simulink model "RoverPlatformArch"  (R2026a)
settings: Solver=VariableStepAuto
settings Model: DataDictionary=RoverPlatformInterfaces.sldd  Creator=potlo  LastModifiedBy=potlo

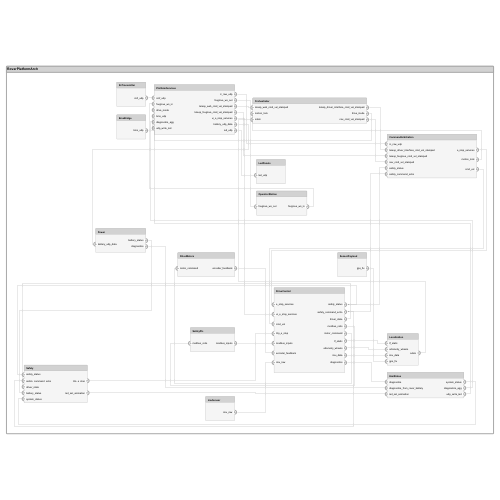
[thumbnail: Simulink's stored preview of the top-level diagram]
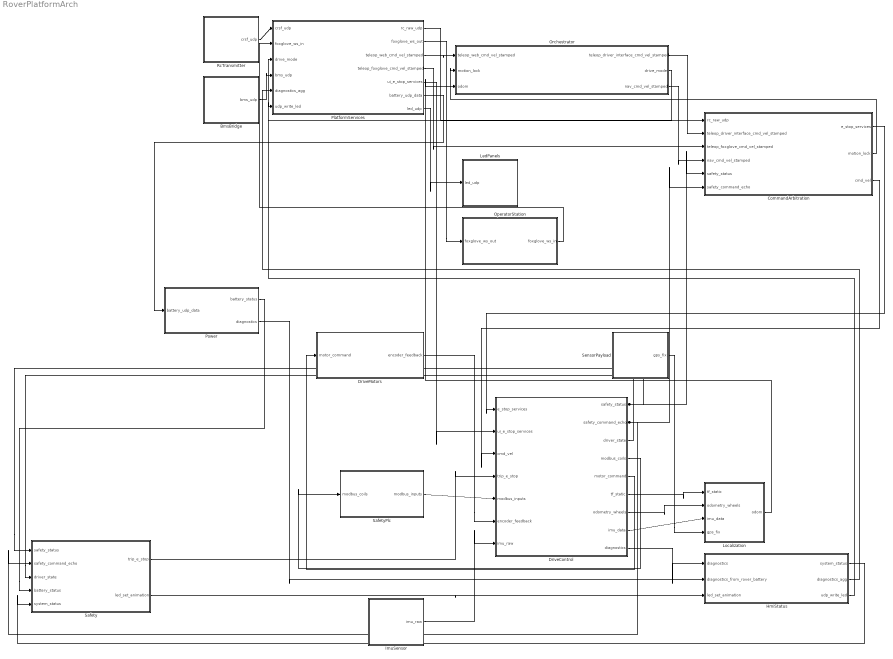
== system RoverPlatformArch ==
  BmsBridge : Subsystem
      settings: PortSchema="{\"entries\":[{\"content\":{\"headerSize\":26,\"margin\":15,\"minimumSpacing\":25,\"sides\":[{\"content\":{},\"type\":\"ConnectorPlacement.EquallySpacedRectSide\",\"uuid\":\"6054c9f0-8412-410d-9e26-05323c576afd\"},{\"content\":{\"connectorIds\":[\"Out1\"],\"side\":\"RIGHT\"},\"type\":\"ConnectorPlacement.EquallySpacedRectSide\",\"uuid\":\"23d80627-c7f5-467f-845e-39a8ba0f8903\"},{\"content\":{\"side\":\"TOP\"},\"type\":\"ConnectorPlacement.EquallySpacedRectSide\",\"uuid\":\"85f79d16-0e4c-46b5-a9e4-5492e918629f\"}]},\"type\":\"ConnectorPlacement.EquallySpacedConnector\",\"uuid\":\"014a8f15-8cf2-4a07-97a2-6bf2fab6c72b\"}],\"packageUris\":[\"http://schema.mathworks.com/mf0/Connector/R2020b\"],\"version\":\"1.0\"}"
  CommandArbitration : Subsystem
      settings: PortSchema="{\"entries\":[{\"content\":{\"headerSize\":26,\"margin\":15,\"minimumSpacing\":25,\"sides\":[{\"content\":{\"connectorIds\":[\"In1\",\"In2\",\"In3\",\"In4\",\"In5\",\"In6\"]},\"type\":\"ConnectorPlacement.EquallySpacedRectSide\",\"uuid\":\"6054c9f0-8412-410d-9e26-05323c576afd\"},{\"content\":{\"connectorIds\":[\"Out1\",\"Out2\",\"Out3\"],\"side\":\"RIGHT\"},\"type\":\"ConnectorPlacement.EquallySpacedRectSide\",\"uuid\":\"23d80627-c7f5-467f-845e-39a8ba0f8903\"},{\"content\":{\"side\":\"TOP\"},\"type\":\"ConnectorPlacement.EquallySpacedRectSide\",\"uuid\":\"85f79d16-0e4c-46b5-a9e4-5492e918629f\"}]},\"type\":\"ConnectorPlacement.EquallySpacedConnector\",\"uuid\":\"014a8f15-8cf2-4a07-97a2-6bf2fab6c72b\"}],\"packageUris\":[\"http://schema.mathworks.com/mf0/Connector/R2020b\"],\"version\":\"1.0\"}"
  DriveControl : Subsystem
      settings: PortSchema="{\"entries\":[{\"content\":{\"headerSize\":26,\"margin\":15,\"minimumSpacing\":25,\"sides\":[{\"content\":{\"connectorIds\":[\"In1\",\"In2\",\"In3\",\"In4\",\"In5\",\"In6\",\"In7\"]},\"type\":\"ConnectorPlacement.EquallySpacedRectSide\",\"uuid\":\"6054c9f0-8412-410d-9e26-05323c576afd\"},{\"content\":{\"connectorIds\":[\"Out1\",\"Out2\",\"Out3\",\"Out4\",\"Out5\",\"Out6\",\"Out7\",\"Out8\",\"Out9\"],\"side\":\"RIGHT\"},\"type\":\"ConnectorPlacement.EquallySpacedRectSide\",\"uuid\":\"23d80627-c7f5-467f-845e-39a8ba0f8903\"},{\"content\":{\"side\":\"TOP\"},\"type\":\"ConnectorPlacement.EquallySpacedRectSide\",\"uuid\":\"85f79d16-0e4c-46b5-a9e4-5492e918629f\"}]},\"type\":\"ConnectorPlacement.EquallySpacedConnector\",\"uuid\":\"014a8f15-8cf2-4a07-97a2-6bf2fab6c72b\"}],\"packageUris\":[\"http://schema.mathworks.com/mf0/Connector/R2020b\"],\"version\":\"1.0\"}"
  DriveMotors : Subsystem
      settings: PortSchema="{\"entries\":[{\"content\":{\"headerSize\":26,\"margin\":15,\"minimumSpacing\":25,\"sides\":[{\"content\":{\"connectorIds\":[\"In1\"]},\"type\":\"ConnectorPlacement.EquallySpacedRectSide\",\"uuid\":\"6054c9f0-8412-410d-9e26-05323c576afd\"},{\"content\":{\"connectorIds\":[\"Out1\"],\"side\":\"RIGHT\"},\"type\":\"ConnectorPlacement.EquallySpacedRectSide\",\"uuid\":\"23d80627-c7f5-467f-845e-39a8ba0f8903\"},{\"content\":{\"side\":\"TOP\"},\"type\":\"ConnectorPlacement.EquallySpacedRectSide\",\"uuid\":\"85f79d16-0e4c-46b5-a9e4-5492e918629f\"}]},\"type\":\"ConnectorPlacement.EquallySpacedConnector\",\"uuid\":\"014a8f15-8cf2-4a07-97a2-6bf2fab6c72b\"}],\"packageUris\":[\"http://schema.mathworks.com/mf0/Connector/R2020b\"],\"version\":\"1.0\"}"
  HmiStatus : Subsystem
      settings: PortSchema="{\"entries\":[{\"content\":{\"headerSize\":26,\"margin\":15,\"minimumSpacing\":25,\"sides\":[{\"content\":{\"connectorIds\":[\"In1\",\"In2\",\"In3\"]},\"type\":\"ConnectorPlacement.EquallySpacedRectSide\",\"uuid\":\"6054c9f0-8412-410d-9e26-05323c576afd\"},{\"content\":{\"connectorIds\":[\"Out1\",\"Out2\",\"Out3\"],\"side\":\"RIGHT\"},\"type\":\"ConnectorPlacement.EquallySpacedRectSide\",\"uuid\":\"23d80627-c7f5-467f-845e-39a8ba0f8903\"},{\"content\":{\"side\":\"TOP\"},\"type\":\"ConnectorPlacement.EquallySpacedRectSide\",\"uuid\":\"85f79d16-0e4c-46b5-a9e4-5492e918629f\"}]},\"type\":\"ConnectorPlacement.EquallySpacedConnector\",\"uuid\":\"014a8f15-8cf2-4a07-97a2-6bf2fab6c72b\"}],\"packageUris\":[\"http://schema.mathworks.com/mf0/Connector/R2020b\"],\"version\":\"1.0\"}"
  ImuSensor : Subsystem
      settings: PortSchema="{\"entries\":[{\"content\":{\"headerSize\":26,\"margin\":15,\"minimumSpacing\":25,\"sides\":[{\"content\":{},\"type\":\"ConnectorPlacement.EquallySpacedRectSide\",\"uuid\":\"6054c9f0-8412-410d-9e26-05323c576afd\"},{\"content\":{\"connectorIds\":[\"Out1\"],\"side\":\"RIGHT\"},\"type\":\"ConnectorPlacement.EquallySpacedRectSide\",\"uuid\":\"23d80627-c7f5-467f-845e-39a8ba0f8903\"},{\"content\":{\"side\":\"TOP\"},\"type\":\"ConnectorPlacement.EquallySpacedRectSide\",\"uuid\":\"85f79d16-0e4c-46b5-a9e4-5492e918629f\"}]},\"type\":\"ConnectorPlacement.EquallySpacedConnector\",\"uuid\":\"014a8f15-8cf2-4a07-97a2-6bf2fab6c72b\"}],\"packageUris\":[\"http://schema.mathworks.com/mf0/Connector/R2020b\"],\"version\":\"1.0\"}"
  LedPanels : Subsystem
      settings: PortSchema="{\"entries\":[{\"content\":{\"headerSize\":26,\"margin\":15,\"minimumSpacing\":25,\"sides\":[{\"content\":{\"connectorIds\":[\"In1\"]},\"type\":\"ConnectorPlacement.EquallySpacedRectSide\",\"uuid\":\"6054c9f0-8412-410d-9e26-05323c576afd\"},{\"content\":{\"side\":\"RIGHT\"},\"type\":\"ConnectorPlacement.EquallySpacedRectSide\",\"uuid\":\"23d80627-c7f5-467f-845e-39a8ba0f8903\"},{\"content\":{\"side\":\"TOP\"},\"type\":\"ConnectorPlacement.EquallySpacedRectSide\",\"uuid\":\"85f79d16-0e4c-46b5-a9e4-5492e918629f\"}]},\"type\":\"ConnectorPlacement.EquallySpacedConnector\",\"uuid\":\"014a8f15-8cf2-4a07-97a2-6bf2fab6c72b\"}],\"packageUris\":[\"http://schema.mathworks.com/mf0/Connector/R2020b\"],\"version\":\"1.0\"}"
  Localization : Subsystem
      settings: PortSchema="{\"entries\":[{\"content\":{\"headerSize\":26,\"margin\":15,\"minimumSpacing\":25,\"sides\":[{\"content\":{\"connectorIds\":[\"In1\",\"In2\",\"In3\",\"In4\"]},\"type\":\"ConnectorPlacement.EquallySpacedRectSide\",\"uuid\":\"6054c9f0-8412-410d-9e26-05323c576afd\"},{\"content\":{\"connectorIds\":[\"Out1\"],\"side\":\"RIGHT\"},\"type\":\"ConnectorPlacement.EquallySpacedRectSide\",\"uuid\":\"23d80627-c7f5-467f-845e-39a8ba0f8903\"},{\"content\":{\"side\":\"TOP\"},\"type\":\"ConnectorPlacement.EquallySpacedRectSide\",\"uuid\":\"85f79d16-0e4c-46b5-a9e4-5492e918629f\"}]},\"type\":\"ConnectorPlacement.EquallySpacedConnector\",\"uuid\":\"014a8f15-8cf2-4a07-97a2-6bf2fab6c72b\"}],\"packageUris\":[\"http://schema.mathworks.com/mf0/Connector/R2020b\"],\"version\":\"1.0\"}"
  OperatorStation : Subsystem
      settings: PortSchema="{\"entries\":[{\"content\":{\"headerSize\":26,\"margin\":15,\"minimumSpacing\":25,\"sides\":[{\"content\":{\"connectorIds\":[\"In1\"]},\"type\":\"ConnectorPlacement.EquallySpacedRectSide\",\"uuid\":\"6054c9f0-8412-410d-9e26-05323c576afd\"},{\"content\":{\"connectorIds\":[\"Out1\"],\"side\":\"RIGHT\"},\"type\":\"ConnectorPlacement.EquallySpacedRectSide\",\"uuid\":\"23d80627-c7f5-467f-845e-39a8ba0f8903\"},{\"content\":{\"side\":\"TOP\"},\"type\":\"ConnectorPlacement.EquallySpacedRectSide\",\"uuid\":\"85f79d16-0e4c-46b5-a9e4-5492e918629f\"}]},\"type\":\"ConnectorPlacement.EquallySpacedConnector\",\"uuid\":\"014a8f15-8cf2-4a07-97a2-6bf2fab6c72b\"}],\"packageUris\":[\"http://schema.mathworks.com/mf0/Connector/R2020b\"],\"version\":\"1.0\"}"
  Orchestrator : Subsystem
      settings: PortSchema="{\"entries\":[{\"content\":{\"headerSize\":26,\"margin\":15,\"minimumSpacing\":25,\"sides\":[{\"content\":{\"connectorIds\":[\"In1\",\"In2\",\"In3\"]},\"type\":\"ConnectorPlacement.EquallySpacedRectSide\",\"uuid\":\"6054c9f0-8412-410d-9e26-05323c576afd\"},{\"content\":{\"connectorIds\":[\"Out1\",\"Out2\",\"Out3\"],\"side\":\"RIGHT\"},\"type\":\"ConnectorPlacement.EquallySpacedRectSide\",\"uuid\":\"23d80627-c7f5-467f-845e-39a8ba0f8903\"},{\"content\":{\"side\":\"TOP\"},\"type\":\"ConnectorPlacement.EquallySpacedRectSide\",\"uuid\":\"85f79d16-0e4c-46b5-a9e4-5492e918629f\"}]},\"type\":\"ConnectorPlacement.EquallySpacedConnector\",\"uuid\":\"014a8f15-8cf2-4a07-97a2-6bf2fab6c72b\"}],\"packageUris\":[\"http://schema.mathworks.com/mf0/Connector/R2020b\"],\"version\":\"1.0\"}"
  PlatformServices : Subsystem
      settings: PortSchema="{\"entries\":[{\"content\":{\"headerSize\":26,\"margin\":15,\"minimumSpacing\":25,\"sides\":[{\"content\":{\"connectorIds\":[\"In1\",\"In2\",\"In3\",\"In4\",\"In5\",\"In6\"]},\"type\":\"ConnectorPlacement.EquallySpacedRectSide\",\"uuid\":\"6054c9f0-8412-410d-9e26-05323c576afd\"},{\"content\":{\"connectorIds\":[\"Out1\",\"Out2\",\"Out3\",\"Out4\",\"Out5\",\"Out6\",\"Out7\"],\"side\":\"RIGHT\"},\"type\":\"ConnectorPlacement.EquallySpacedRectSide\",\"uuid\":\"23d80627-c7f5-467f-845e-39a8ba0f8903\"},{\"content\":{\"side\":\"TOP\"},\"type\":\"ConnectorPlacement.EquallySpacedRectSide\",\"uuid\":\"85f79d16-0e4c-46b5-a9e4-5492e918629f\"}]},\"type\":\"ConnectorPlacement.EquallySpacedConnector\",\"uuid\":\"014a8f15-8cf2-4a07-97a2-6bf2fab6c72b\"}],\"packageUris\":[\"http://schema.mathworks.com/mf0/Connector/R2020b\"],\"version\":\"1.0\"}"
  Power : Subsystem
      settings: PortSchema="{\"entries\":[{\"content\":{\"headerSize\":26,\"margin\":15,\"minimumSpacing\":25,\"sides\":[{\"content\":{\"connectorIds\":[\"In1\"]},\"type\":\"ConnectorPlacement.EquallySpacedRectSide\",\"uuid\":\"6054c9f0-8412-410d-9e26-05323c576afd\"},{\"content\":{\"connectorIds\":[\"Out1\",\"Out2\"],\"side\":\"RIGHT\"},\"type\":\"ConnectorPlacement.EquallySpacedRectSide\",\"uuid\":\"23d80627-c7f5-467f-845e-39a8ba0f8903\"},{\"content\":{\"side\":\"TOP\"},\"type\":\"ConnectorPlacement.EquallySpacedRectSide\",\"uuid\":\"85f79d16-0e4c-46b5-a9e4-5492e918629f\"}]},\"type\":\"ConnectorPlacement.EquallySpacedConnector\",\"uuid\":\"014a8f15-8cf2-4a07-97a2-6bf2fab6c72b\"}],\"packageUris\":[\"http://schema.mathworks.com/mf0/Connector/R2020b\"],\"version\":\"1.0\"}"
  RcTransmitter : Subsystem
      settings: PortSchema="{\"entries\":[{\"content\":{\"headerSize\":26,\"margin\":15,\"minimumSpacing\":25,\"sides\":[{\"content\":{},\"type\":\"ConnectorPlacement.EquallySpacedRectSide\",\"uuid\":\"6054c9f0-8412-410d-9e26-05323c576afd\"},{\"content\":{\"connectorIds\":[\"Out1\"],\"side\":\"RIGHT\"},\"type\":\"ConnectorPlacement.EquallySpacedRectSide\",\"uuid\":\"23d80627-c7f5-467f-845e-39a8ba0f8903\"},{\"content\":{\"side\":\"TOP\"},\"type\":\"ConnectorPlacement.EquallySpacedRectSide\",\"uuid\":\"85f79d16-0e4c-46b5-a9e4-5492e918629f\"}]},\"type\":\"ConnectorPlacement.EquallySpacedConnector\",\"uuid\":\"014a8f15-8cf2-4a07-97a2-6bf2fab6c72b\"}],\"packageUris\":[\"http://schema.mathworks.com/mf0/Connector/R2020b\"],\"version\":\"1.0\"}"
  Safety : Subsystem
      settings: PortSchema="{\"entries\":[{\"content\":{\"headerSize\":26,\"margin\":15,\"minimumSpacing\":25,\"sides\":[{\"content\":{\"connectorIds\":[\"In1\",\"In2\",\"In3\",\"In4\",\"In5\"]},\"type\":\"ConnectorPlacement.EquallySpacedRectSide\",\"uuid\":\"6054c9f0-8412-410d-9e26-05323c576afd\"},{\"content\":{\"connectorIds\":[\"Out1\",\"Out2\"],\"side\":\"RIGHT\"},\"type\":\"ConnectorPlacement.EquallySpacedRectSide\",\"uuid\":\"23d80627-c7f5-467f-845e-39a8ba0f8903\"},{\"content\":{\"side\":\"TOP\"},\"type\":\"ConnectorPlacement.EquallySpacedRectSide\",\"uuid\":\"85f79d16-0e4c-46b5-a9e4-5492e918629f\"}]},\"type\":\"ConnectorPlacement.EquallySpacedConnector\",\"uuid\":\"014a8f15-8cf2-4a07-97a2-6bf2fab6c72b\"}],\"packageUris\":[\"http://schema.mathworks.com/mf0/Connector/R2020b\"],\"version\":\"1.0\"}"
  SafetyPlc : Subsystem
      settings: PortSchema="{\"entries\":[{\"content\":{\"headerSize\":26,\"margin\":15,\"minimumSpacing\":25,\"sides\":[{\"content\":{\"connectorIds\":[\"In1\"]},\"type\":\"ConnectorPlacement.EquallySpacedRectSide\",\"uuid\":\"6054c9f0-8412-410d-9e26-05323c576afd\"},{\"content\":{\"connectorIds\":[\"Out1\"],\"side\":\"RIGHT\"},\"type\":\"ConnectorPlacement.EquallySpacedRectSide\",\"uuid\":\"23d80627-c7f5-467f-845e-39a8ba0f8903\"},{\"content\":{\"side\":\"TOP\"},\"type\":\"ConnectorPlacement.EquallySpacedRectSide\",\"uuid\":\"85f79d16-0e4c-46b5-a9e4-5492e918629f\"}]},\"type\":\"ConnectorPlacement.EquallySpacedConnector\",\"uuid\":\"014a8f15-8cf2-4a07-97a2-6bf2fab6c72b\"}],\"packageUris\":[\"http://schema.mathworks.com/mf0/Connector/R2020b\"],\"version\":\"1.0\"}"
  SensorPayload : Subsystem
      settings: PortSchema="{\"entries\":[{\"content\":{\"headerSize\":26,\"margin\":15,\"minimumSpacing\":25,\"sides\":[{\"content\":{},\"type\":\"ConnectorPlacement.EquallySpacedRectSide\",\"uuid\":\"6054c9f0-8412-410d-9e26-05323c576afd\"},{\"content\":{\"connectorIds\":[\"Out1\"],\"side\":\"RIGHT\"},\"type\":\"ConnectorPlacement.EquallySpacedRectSide\",\"uuid\":\"23d80627-c7f5-467f-845e-39a8ba0f8903\"},{\"content\":{\"side\":\"TOP\"},\"type\":\"ConnectorPlacement.EquallySpacedRectSide\",\"uuid\":\"85f79d16-0e4c-46b5-a9e4-5492e918629f\"}]},\"type\":\"ConnectorPlacement.EquallySpacedConnector\",\"uuid\":\"014a8f15-8cf2-4a07-97a2-6bf2fab6c72b\"}],\"packageUris\":[\"http://schema.mathworks.com/mf0/Connector/R2020b\"],\"version\":\"1.0\"}"
  wires:
  PlatformServices/4(teleop_foxglove_cmd_vel_stamped) -> CommandArbitration/3(teleop_foxglove_cmd_vel_stamped)
  RcTransmitter/1(crsf_udp) -> PlatformServices/1(crsf_udp)
  Power/1(battery_status) -> Safety/4(battery_status)
  HmiStatus/1(system_status) -> Safety/5(system_status)
  Safety/1(trip_e_stop) -> DriveControl/4(trip_e_stop)
  Power/2(diagnostics) -> HmiStatus/2(diagnostics_from_rover_battery)
  Safety/2(led_set_animation) -> HmiStatus/3(led_set_animation)
  BmsBridge/1(bms_udp) -> PlatformServices/4(bms_udp)
  PlatformServices/1(rc_raw_udp) -> CommandArbitration/1(rc_raw_udp)
  DriveControl/7(odometry_wheels) -> Localization/2(odometry_wheels)
  PlatformServices/2(foxglove_ws_out) -> OperatorStation/1(foxglove_ws_out)
  PlatformServices/3(teleop_web_cmd_vel_stamped) -> Orchestrator/1(teleop_web_cmd_vel_stamped)
  PlatformServices/5(ui_e_stop_services) -> DriveControl/2(ui_e_stop_services)
  PlatformServices/6(battery_udp_data) -> Power/1(battery_udp_data)
  PlatformServices/7(led_udp) -> LedPanels/1(led_udp)
  DriveMotors/1(encoder_feedback) -> DriveControl/6(encoder_feedback)
  SafetyPlc/1(modbus_inputs) -> DriveControl/5(modbus_inputs)
  DriveControl/1(safety_status) -> Safety/1(safety_status), CommandArbitration/5(safety_status)
  ImuSensor/1(imu_raw) -> DriveControl/7(imu_raw)
  SensorPayload/1(gps_fix) -> Localization/4(gps_fix)
  Orchestrator/1(teleop_driver_interface_cmd_vel_stamped) -> CommandArbitration/2(teleop_driver_interface_cmd_vel_stamped)
  Localization/1(odom) -> Orchestrator/3(odom)
  Orchestrator/2(drive_mode) -> PlatformServices/3(drive_mode)
  Orchestrator/3(nav_cmd_vel_stamped) -> CommandArbitration/4(nav_cmd_vel_stamped)
  OperatorStation/1(foxglove_ws_in) -> PlatformServices/2(foxglove_ws_in)
  DriveControl/2(safety_command_echo) -> CommandArbitration/6(safety_command_echo), Safety/2(safety_command_echo)
  DriveControl/3(driver_state) -> Safety/3(driver_state)
  DriveControl/4(modbus_coils) -> SafetyPlc/1(modbus_coils)
  HmiStatus/3(udp_write_led) -> PlatformServices/6(udp_write_led)
  DriveControl/5(motor_command) -> DriveMotors/1(motor_command)
  DriveControl/6(tf_static) -> Localization/1(tf_static)
  DriveControl/8(imu_data) -> Localization/3(imu_data)
  DriveControl/9(diagnostics) -> HmiStatus/1(diagnostics)
  CommandArbitration/1(e_stop_services) -> DriveControl/1(e_stop_services)
  CommandArbitration/2(motion_lock) -> Orchestrator/2(motion_lock)
  CommandArbitration/3(cmd_vel) -> DriveControl/3(cmd_vel)
  HmiStatus/2(diagnostics_agg) -> PlatformServices/5(diagnostics_agg)

== system RoverPlatformArch/BmsBridge ==
  Bus Element Out1 : Outport  PortName=bms_udp

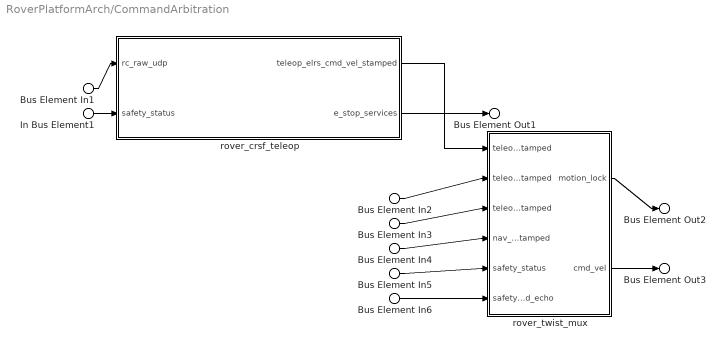
== system RoverPlatformArch/CommandArbitration ==
  Bus Element In1 : Inport  PortName=rc_raw_udp
  Bus Element In2 : Inport  Port=2  PortName=teleop_driver_interface_cmd_vel_stamped
  Bus Element In3 : Inport  Port=3  PortName=teleop_foxglove_cmd_vel_stamped
  Bus Element In4 : Inport  Port=4  PortName=nav_cmd_vel_stamped
  Bus Element In5 : Inport  Port=5  PortName=safety_status
  In Bus Element1 : Inport  Port=5  PortName=safety_status
  Bus Element In6 : Inport  Port=6  PortName=safety_command_echo
  rover_crsf_teleop : Subsystem
      settings: PortSchema="{\"entries\":[{\"content\":{\"headerSize\":26,\"margin\":15,\"minimumSpacing\":25,\"sides\":[{\"content\":{\"connectorIds\":[\"In1\",\"In2\"]},\"type\":\"ConnectorPlacement.EquallySpacedRectSide\",\"uuid\":\"6054c9f0-8412-410d-9e26-05323c576afd\"},{\"content\":{\"connectorIds\":[\"Out1\",\"Out2\"],\"side\":\"RIGHT\"},\"type\":\"ConnectorPlacement.EquallySpacedRectSide\",\"uuid\":\"23d80627-c7f5-467f-845e-39a8ba0f8903\"},{\"content\":{\"side\":\"TOP\"},\"type\":\"ConnectorPlacement.EquallySpacedRectSide\",\"uuid\":\"85f79d16-0e4c-46b5-a9e4-5492e918629f\"}]},\"type\":\"ConnectorPlacement.EquallySpacedConnector\",\"uuid\":\"014a8f15-8cf2-4a07-97a2-6bf2fab6c72b\"}],\"packageUris\":[\"http://schema.mathworks.com/mf0/Connector/R2020b\"],\"version\":\"1.0\"}"
  rover_twist_mux : Subsystem  mask{prio_nav=5, timeout_nav=0.5, prio_driver_interface=8, timeout_driver_interface=0.3, prio_joystick=100, timeout_joystick=0.5, prio_elrs=110, timeout_elrs=0.5, prio_motion_lock=200, timeout_motion_lock=0.5, motion_lock_rate=10, motion_lock_gpio_timeout=1}
      settings: PortSchema="{\"entries\":[{\"content\":{\"headerSize\":26,\"margin\":15,\"minimumSpacing\":25,\"sides\":[{\"content\":{\"connectorIds\":[\"In1\",\"In2\",\"In3\",\"In4\",\"In5\",\"In6\"]},\"type\":\"ConnectorPlacement.EquallySpacedRectSide\",\"uuid\":\"6054c9f0-8412-410d-9e26-05323c576afd\"},{\"content\":{\"connectorIds\":[\"Out1\",\"Out2\"],\"side\":\"RIGHT\"},\"type\":\"ConnectorPlacement.EquallySpacedRectSide\",\"uuid\":\"23d80627-c7f5-467f-845e-39a8ba0f8903\"},{\"content\":{\"side\":\"TOP\"},\"type\":\"ConnectorPlacement.EquallySpacedRectSide\",\"uuid\":\"85f79d16-0e4c-46b5-a9e4-5492e918629f\"}]},\"type\":\"ConnectorPlacement.EquallySpacedConnector\",\"uuid\":\"014a8f15-8cf2-4a07-97a2-6bf2fab6c72b\"}],\"packageUris\":[\"http://schema.mathworks.com/mf0/Connector/R2020b\"],\"version\":\"1.0\"}"
  Bus Element Out1 : Outport  PortName=e_stop_services
  Bus Element Out2 : Outport  Port=2  PortName=motion_lock
  Bus Element Out3 : Outport  Port=3  PortName=cmd_vel
  wires:
  In Bus Element1/1 -> rover_crsf_teleop/2(safety_status)
  Bus Element In1/1 -> rover_crsf_teleop/1(rc_raw_udp)
  Bus Element In5/1 -> rover_twist_mux/5(safety_status)
  rover_crsf_teleop/2(e_stop_services) -> Bus Element Out1/1
  rover_crsf_teleop/1(teleop_elrs_cmd_vel_stamped) -> rover_twist_mux/1(teleop_elrs_cmd_vel_stamped)
  Bus Element In3/1 -> rover_twist_mux/3(teleop_foxglove_cmd_vel_stamped)
  Bus Element In2/1 -> rover_twist_mux/2(teleop_driver_interface_cmd_vel_stamped)
  Bus Element In4/1 -> rover_twist_mux/4(nav_cmd_vel_stamped)
  Bus Element In6/1 -> rover_twist_mux/6(safety_command_echo)
  rover_twist_mux/1(motion_lock) -> Bus Element Out2/1
  rover_twist_mux/2(cmd_vel) -> Bus Element Out3/1

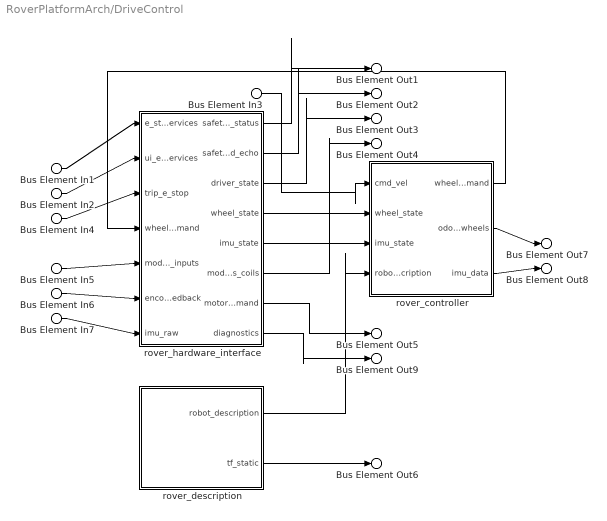
== system RoverPlatformArch/DriveControl ==
  Bus Element In1 : Inport  PortName=e_stop_services
  Bus Element In2 : Inport  Port=2  PortName=ui_e_stop_services
  Bus Element In3 : Inport  Port=3  PortName=cmd_vel
  Bus Element In4 : Inport  Port=4  PortName=trip_e_stop
  Bus Element In5 : Inport  Port=5  PortName=modbus_inputs
  Bus Element In6 : Inport  Port=6  PortName=encoder_feedback
  Bus Element In7 : Inport  Port=7  PortName=imu_raw
  rover_controller : Subsystem  mask{cm_update_rate=100, diff_drive_update_rate=50, imu_broadcaster_rate=50, joint_state_rate=20, wheel_separation=0.617, wheel_radius=0.1651, wheel_separation_multiplier=1.659, cmd_vel_timeout=0.5, max_linear_velocity=0.95, max_linear_acceleration=2.7, max_angular_velocity=1.5, max_angular_acceleration=3.74}
      settings: PortSchema="{\"entries\":[{\"content\":{\"headerSize\":26,\"margin\":15,\"minimumSpacing\":25,\"sides\":[{\"content\":{\"connectorIds\":[\"In1\",\"In2\",\"In3\",\"In4\"]},\"type\":\"ConnectorPlacement.EquallySpacedRectSide\",\"uuid\":\"6054c9f0-8412-410d-9e26-05323c576afd\"},{\"content\":{\"connectorIds\":[\"Out1\",\"Out2\",\"Out3\"],\"side\":\"RIGHT\"},\"type\":\"ConnectorPlacement.EquallySpacedRectSide\",\"uuid\":\"23d80627-c7f5-467f-845e-39a8ba0f8903\"},{\"content\":{\"side\":\"TOP\"},\"type\":\"ConnectorPlacement.EquallySpacedRectSide\",\"uuid\":\"85f79d16-0e4c-46b5-a9e4-5492e918629f\"}]},\"type\":\"ConnectorPlacement.EquallySpacedConnector\",\"uuid\":\"014a8f15-8cf2-4a07-97a2-6bf2fab6c72b\"}],\"packageUris\":[\"http://schema.mathworks.com/mf0/Connector/R2020b\"],\"version\":\"1.0\"}"
  rover_description : Subsystem  mask{wheelbase=0.503, wheel_width=0.108, wheel_mass=4.79294, tyre_radius=0.1699, tyre_y_offset=-0.00171, wheel_mount_point_z=0.037363, body_mass=39.5026, wheel_joint_velocity_limit=10.958}
      settings: PortSchema="{\"entries\":[{\"content\":{\"headerSize\":26,\"margin\":15,\"minimumSpacing\":25,\"sides\":[{\"content\":{},\"type\":\"ConnectorPlacement.EquallySpacedRectSide\",\"uuid\":\"6054c9f0-8412-410d-9e26-05323c576afd\"},{\"content\":{\"connectorIds\":[\"Out1\",\"Out2\"],\"side\":\"RIGHT\"},\"type\":\"ConnectorPlacement.EquallySpacedRectSide\",\"uuid\":\"23d80627-c7f5-467f-845e-39a8ba0f8903\"},{\"content\":{\"side\":\"TOP\"},\"type\":\"ConnectorPlacement.EquallySpacedRectSide\",\"uuid\":\"85f79d16-0e4c-46b5-a9e4-5492e918629f\"}]},\"type\":\"ConnectorPlacement.EquallySpacedConnector\",\"uuid\":\"014a8f15-8cf2-4a07-97a2-6bf2fab6c72b\"}],\"packageUris\":[\"http://schema.mathworks.com/mf0/Connector/R2020b\"],\"version\":\"1.0\"}"
  rover_hardware_interface : Subsystem  mask{modbus_response_timeout=0.15, safety_wdg_kick_period=0.2, safety_io_poll_period=0.1, safety_latch_reset_pulse=0.1, driver_states_update_frequency=20, driver_comm_timeout=0.3, motor_failsafe_timeout=0.5, motor_current_limit=15, gear_ratio=23.3, velocity_command_zero_tolerance=0.4, velocity_state_zero_tolerance=0.05, contactor_dropout_tolerance=0.5, imu_data_interval=0.008}
      settings: PortSchema="{\"entries\":[{\"content\":{\"headerSize\":26,\"margin\":15,\"minimumSpacing\":25,\"sides\":[{\"content\":{\"connectorIds\":[\"In1\",\"In2\",\"In3\",\"In4\",\"In5\",\"In6\",\"In7\"]},\"type\":\"ConnectorPlacement.EquallySpacedRectSide\",\"uuid\":\"6054c9f0-8412-410d-9e26-05323c576afd\"},{\"content\":{\"connectorIds\":[\"Out1\",\"Out2\",\"Out3\",\"Out4\",\"Out5\",\"Out6\",\"Out7\",\"Out8\"],\"side\":\"RIGHT\"},\"type\":\"ConnectorPlacement.EquallySpacedRectSide\",\"uuid\":\"23d80627-c7f5-467f-845e-39a8ba0f8903\"},{\"content\":{\"side\":\"TOP\"},\"type\":\"ConnectorPlacement.EquallySpacedRectSide\",\"uuid\":\"85f79d16-0e4c-46b5-a9e4-5492e918629f\"}]},\"type\":\"ConnectorPlacement.EquallySpacedConnector\",\"uuid\":\"014a8f15-8cf2-4a07-97a2-6bf2fab6c72b\"}],\"packageUris\":[\"http://schema.mathworks.com/mf0/Connector/R2020b\"],\"version\":\"1.0\"}"
  Bus Element Out1 : Outport  PortName=safety_status
  Bus Element Out2 : Outport  Port=2  PortName=safety_command_echo
  Bus Element Out3 : Outport  Port=3  PortName=driver_state
  Bus Element Out4 : Outport  Port=4  PortName=modbus_coils
  Bus Element Out5 : Outport  Port=5  PortName=motor_command
  Bus Element Out6 : Outport  Port=6  PortName=tf_static
  Bus Element Out7 : Outport  Port=7  PortName=odometry_wheels
  Bus Element Out8 : Outport  Port=8  PortName=imu_data
  Bus Element Out9 : Outport  Port=9  PortName=diagnostics
  wires:
  Bus Element In5/1 -> rover_hardware_interface/5(modbus_inputs)
  Bus Element In1/1 -> rover_hardware_interface/1(e_stop_services)
  Bus Element In4/1 -> rover_hardware_interface/3(trip_e_stop)
  rover_hardware_interface/6(modbus_coils) -> Bus Element Out4/1
  Bus Element In2/1 -> rover_hardware_interface/2(ui_e_stop_services)
  rover_hardware_interface/1(safety_status) -> Bus Element Out1/1
  Bus Element In7/1 -> rover_hardware_interface/7(imu_raw)
  Bus Element In3/1 -> rover_controller/1(cmd_vel)
  rover_description/2(tf_static) -> Bus Element Out6/1
  Bus Element In6/1 -> rover_hardware_interface/6(encoder_feedback)
  rover_hardware_interface/2(safety_command_echo) -> Bus Element Out2/1
  rover_hardware_interface/3(driver_state) -> Bus Element Out3/1
  rover_hardware_interface/8(diagnostics) -> Bus Element Out9/1
  rover_hardware_interface/4(wheel_state) -> rover_controller/2(wheel_state)
  rover_hardware_interface/5(imu_state) -> rover_controller/3(imu_state)
  rover_hardware_interface/7(motor_command) -> Bus Element Out5/1
  rover_description/1(robot_description) -> rover_controller/4(robot_description)
  rover_controller/1(wheel_velocity_command) -> rover_hardware_interface/4(wheel_velocity_command)
  rover_controller/2(odometry_wheels) -> Bus Element Out7/1
  rover_controller/3(imu_data) -> Bus Element Out8/1

== system RoverPlatformArch/DriveMotors ==
  Bus Element In1 : Inport  PortName=motor_command
  Bus Element Out1 : Outport  PortName=encoder_feedback

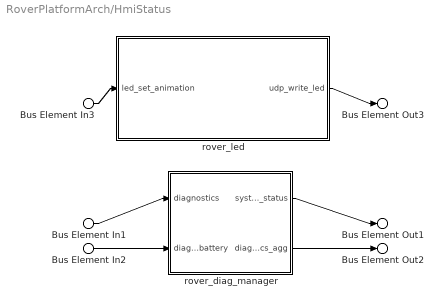
== system RoverPlatformArch/HmiStatus ==
  Bus Element In1 : Inport  PortName=diagnostics
  Bus Element In2 : Inport  Port=2  PortName=diagnostics_from_rover_battery
  Bus Element In3 : Inport  Port=3  PortName=led_set_animation
  rover_diag_manager : Subsystem  mask{system_status_rate=5, diagnostics_agg_rate=1}
      settings: PortSchema="{\"entries\":[{\"content\":{\"headerSize\":26,\"margin\":15,\"minimumSpacing\":25,\"sides\":[{\"content\":{\"connectorIds\":[\"In1\",\"In2\"]},\"type\":\"ConnectorPlacement.EquallySpacedRectSide\",\"uuid\":\"6054c9f0-8412-410d-9e26-05323c576afd\"},{\"content\":{\"connectorIds\":[\"Out1\",\"Out2\"],\"side\":\"RIGHT\"},\"type\":\"ConnectorPlacement.EquallySpacedRectSide\",\"uuid\":\"23d80627-c7f5-467f-845e-39a8ba0f8903\"},{\"content\":{\"side\":\"TOP\"},\"type\":\"ConnectorPlacement.EquallySpacedRectSide\",\"uuid\":\"85f79d16-0e4c-46b5-a9e4-5492e918629f\"}]},\"type\":\"ConnectorPlacement.EquallySpacedConnector\",\"uuid\":\"014a8f15-8cf2-4a07-97a2-6bf2fab6c72b\"}],\"packageUris\":[\"http://schema.mathworks.com/mf0/Connector/R2020b\"],\"version\":\"1.0\"}"
  rover_led : Subsystem
      settings: PortSchema="{\"entries\":[{\"content\":{\"headerSize\":26,\"margin\":15,\"minimumSpacing\":25,\"sides\":[{\"content\":{\"connectorIds\":[\"In1\"]},\"type\":\"ConnectorPlacement.EquallySpacedRectSide\",\"uuid\":\"6054c9f0-8412-410d-9e26-05323c576afd\"},{\"content\":{\"connectorIds\":[\"Out1\"],\"side\":\"RIGHT\"},\"type\":\"ConnectorPlacement.EquallySpacedRectSide\",\"uuid\":\"23d80627-c7f5-467f-845e-39a8ba0f8903\"},{\"content\":{\"side\":\"TOP\"},\"type\":\"ConnectorPlacement.EquallySpacedRectSide\",\"uuid\":\"85f79d16-0e4c-46b5-a9e4-5492e918629f\"}]},\"type\":\"ConnectorPlacement.EquallySpacedConnector\",\"uuid\":\"014a8f15-8cf2-4a07-97a2-6bf2fab6c72b\"}],\"packageUris\":[\"http://schema.mathworks.com/mf0/Connector/R2020b\"],\"version\":\"1.0\"}"
  Bus Element Out1 : Outport  PortName=system_status
  Bus Element Out2 : Outport  Port=2  PortName=diagnostics_agg
  Bus Element Out3 : Outport  Port=3  PortName=udp_write_led
  wires:
  Bus Element In2/1 -> rover_diag_manager/2(diagnostics_from_rover_battery)
  Bus Element In1/1 -> rover_diag_manager/1(diagnostics)
  Bus Element In3/1 -> rover_led/1(led_set_animation)
  rover_led/1(udp_write_led) -> Bus Element Out3/1
  rover_diag_manager/1(system_status) -> Bus Element Out1/1
  rover_diag_manager/2(diagnostics_agg) -> Bus Element Out2/1

== system RoverPlatformArch/ImuSensor ==
  Bus Element Out1 : Outport  PortName=imu_raw

== system RoverPlatformArch/LedPanels ==
  Bus Element In1 : Inport  PortName=led_udp

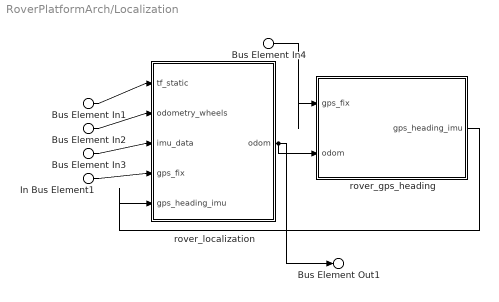
== system RoverPlatformArch/Localization ==
  Bus Element In1 : Inport  PortName=tf_static
  Bus Element In2 : Inport  Port=2  PortName=odometry_wheels
  Bus Element In3 : Inport  Port=3  PortName=imu_data
  Bus Element In4 : Inport  Port=4  PortName=gps_fix
  In Bus Element1 : Inport  Port=4  PortName=gps_fix
  rover_gps_heading : Subsystem
      settings: PortSchema="{\"entries\":[{\"content\":{\"headerSize\":26,\"margin\":15,\"minimumSpacing\":25,\"sides\":[{\"content\":{\"connectorIds\":[\"In1\",\"In2\"]},\"type\":\"ConnectorPlacement.EquallySpacedRectSide\",\"uuid\":\"6054c9f0-8412-410d-9e26-05323c576afd\"},{\"content\":{\"connectorIds\":[\"Out1\"],\"side\":\"RIGHT\"},\"type\":\"ConnectorPlacement.EquallySpacedRectSide\",\"uuid\":\"23d80627-c7f5-467f-845e-39a8ba0f8903\"},{\"content\":{\"side\":\"TOP\"},\"type\":\"ConnectorPlacement.EquallySpacedRectSide\",\"uuid\":\"85f79d16-0e4c-46b5-a9e4-5492e918629f\"}]},\"type\":\"ConnectorPlacement.EquallySpacedConnector\",\"uuid\":\"014a8f15-8cf2-4a07-97a2-6bf2fab6c72b\"}],\"packageUris\":[\"http://schema.mathworks.com/mf0/Connector/R2020b\"],\"version\":\"1.0\"}"
  rover_localization : Subsystem  mask{ekf_frequency=50}
      settings: PortSchema="{\"entries\":[{\"content\":{\"headerSize\":26,\"margin\":15,\"minimumSpacing\":25,\"sides\":[{\"content\":{\"connectorIds\":[\"In1\",\"In2\",\"In3\",\"In4\",\"In5\"]},\"type\":\"ConnectorPlacement.EquallySpacedRectSide\",\"uuid\":\"6054c9f0-8412-410d-9e26-05323c576afd\"},{\"content\":{\"connectorIds\":[\"Out1\"],\"side\":\"RIGHT\"},\"type\":\"ConnectorPlacement.EquallySpacedRectSide\",\"uuid\":\"23d80627-c7f5-467f-845e-39a8ba0f8903\"},{\"content\":{\"side\":\"TOP\"},\"type\":\"ConnectorPlacement.EquallySpacedRectSide\",\"uuid\":\"85f79d16-0e4c-46b5-a9e4-5492e918629f\"}]},\"type\":\"ConnectorPlacement.EquallySpacedConnector\",\"uuid\":\"014a8f15-8cf2-4a07-97a2-6bf2fab6c72b\"}],\"packageUris\":[\"http://schema.mathworks.com/mf0/Connector/R2020b\"],\"version\":\"1.0\"}"
  Bus Element Out1 : Outport  PortName=odom
  wires:
  Bus Element In2/1 -> rover_localization/2(odometry_wheels)
  Bus Element In1/1 -> rover_localization/1(tf_static)
  rover_localization/1(odom) -> rover_gps_heading/2(odom), Bus Element Out1/1
  Bus Element In4/1 -> rover_gps_heading/1(gps_fix)
  In Bus Element1/1 -> rover_localization/4(gps_fix)
  Bus Element In3/1 -> rover_localization/3(imu_data)
  rover_gps_heading/1(gps_heading_imu) -> rover_localization/5(gps_heading_imu)

== system RoverPlatformArch/OperatorStation ==
  Bus Element In1 : Inport  PortName=foxglove_ws_out
  Bus Element Out1 : Outport  PortName=foxglove_ws_in

== system RoverPlatformArch/Orchestrator ==
  Bus Element In1 : Inport  PortName=teleop_web_cmd_vel_stamped
  Bus Element In2 : Inport  Port=2  PortName=motion_lock
  Bus Element In3 : Inport  Port=3  PortName=odom
  Bus Element Out1 : Outport  PortName=teleop_driver_interface_cmd_vel_stamped
  Bus Element Out2 : Outport  Port=2  PortName=drive_mode
  Bus Element Out3 : Outport  Port=3  PortName=nav_cmd_vel_stamped

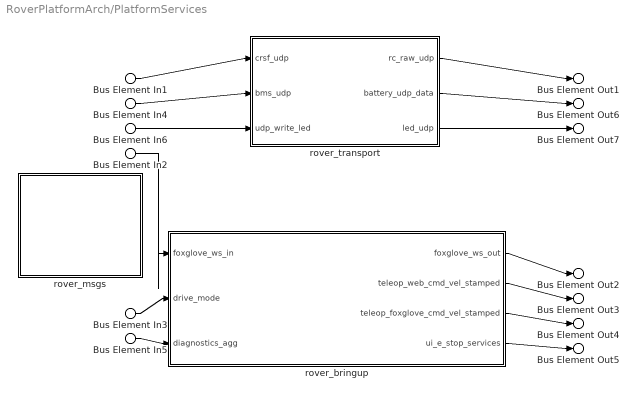
== system RoverPlatformArch/PlatformServices ==
  Bus Element In1 : Inport  PortName=crsf_udp
  Bus Element In2 : Inport  Port=2  PortName=foxglove_ws_in
  Bus Element In3 : Inport  Port=3  PortName=drive_mode
  Bus Element In4 : Inport  Port=4  PortName=bms_udp
  Bus Element In5 : Inport  Port=5  PortName=diagnostics_agg
  Bus Element In6 : Inport  Port=6  PortName=udp_write_led
  rover_bringup : Subsystem
      settings: PortSchema="{\"entries\":[{\"content\":{\"headerSize\":26,\"margin\":15,\"minimumSpacing\":25,\"sides\":[{\"content\":{\"connectorIds\":[\"In1\",\"In2\",\"In3\"]},\"type\":\"ConnectorPlacement.EquallySpacedRectSide\",\"uuid\":\"6054c9f0-8412-410d-9e26-05323c576afd\"},{\"content\":{\"connectorIds\":[\"Out1\",\"Out2\",\"Out3\",\"Out4\"],\"side\":\"RIGHT\"},\"type\":\"ConnectorPlacement.EquallySpacedRectSide\",\"uuid\":\"23d80627-c7f5-467f-845e-39a8ba0f8903\"},{\"content\":{\"side\":\"TOP\"},\"type\":\"ConnectorPlacement.EquallySpacedRectSide\",\"uuid\":\"85f79d16-0e4c-46b5-a9e4-5492e918629f\"}]},\"type\":\"ConnectorPlacement.EquallySpacedConnector\",\"uuid\":\"014a8f15-8cf2-4a07-97a2-6bf2fab6c72b\"}],\"packageUris\":[\"http://schema.mathworks.com/mf0/Connector/R2020b\"],\"version\":\"1.0\"}"
  rover_msgs : Subsystem
      settings: PortSchema="{\"entries\":[{\"content\":{\"headerSize\":26,\"margin\":15,\"minimumSpacing\":25,\"sides\":[{\"content\":{},\"type\":\"ConnectorPlacement.EquallySpacedRectSide\",\"uuid\":\"6054c9f0-8412-410d-9e26-05323c576afd\"},{\"content\":{\"side\":\"RIGHT\"},\"type\":\"ConnectorPlacement.EquallySpacedRectSide\",\"uuid\":\"23d80627-c7f5-467f-845e-39a8ba0f8903\"},{\"content\":{\"side\":\"TOP\"},\"type\":\"ConnectorPlacement.EquallySpacedRectSide\",\"uuid\":\"85f79d16-0e4c-46b5-a9e4-5492e918629f\"}]},\"type\":\"ConnectorPlacement.EquallySpacedConnector\",\"uuid\":\"014a8f15-8cf2-4a07-97a2-6bf2fab6c72b\"}],\"packageUris\":[\"http://schema.mathworks.com/mf0/Connector/R2020b\"],\"version\":\"1.0\"}"
  rover_transport : Subsystem
      settings: PortSchema="{\"entries\":[{\"content\":{\"headerSize\":26,\"margin\":15,\"minimumSpacing\":25,\"sides\":[{\"content\":{\"connectorIds\":[\"In1\",\"In2\",\"In3\"]},\"type\":\"ConnectorPlacement.EquallySpacedRectSide\",\"uuid\":\"6054c9f0-8412-410d-9e26-05323c576afd\"},{\"content\":{\"connectorIds\":[\"Out1\",\"Out2\",\"Out3\"],\"side\":\"RIGHT\"},\"type\":\"ConnectorPlacement.EquallySpacedRectSide\",\"uuid\":\"23d80627-c7f5-467f-845e-39a8ba0f8903\"},{\"content\":{\"side\":\"TOP\"},\"type\":\"ConnectorPlacement.EquallySpacedRectSide\",\"uuid\":\"85f79d16-0e4c-46b5-a9e4-5492e918629f\"}]},\"type\":\"ConnectorPlacement.EquallySpacedConnector\",\"uuid\":\"014a8f15-8cf2-4a07-97a2-6bf2fab6c72b\"}],\"packageUris\":[\"http://schema.mathworks.com/mf0/Connector/R2020b\"],\"version\":\"1.0\"}"
  Bus Element Out1 : Outport  PortName=rc_raw_udp
  Bus Element Out2 : Outport  Port=2  PortName=foxglove_ws_out
  Bus Element Out3 : Outport  Port=3  PortName=teleop_web_cmd_vel_stamped
  Bus Element Out4 : Outport  Port=4  PortName=teleop_foxglove_cmd_vel_stamped
  Bus Element Out5 : Outport  Port=5  PortName=ui_e_stop_services
  Bus Element Out6 : Outport  Port=6  PortName=battery_udp_data
  Bus Element Out7 : Outport  Port=7  PortName=led_udp
  wires:
  rover_transport/2(battery_udp_data) -> Bus Element Out6/1
  Bus Element In3/1 -> rover_bringup/2(drive_mode)
  Bus Element In4/1 -> rover_transport/2(bms_udp)
  Bus Element In1/1 -> rover_transport/1(crsf_udp)
  Bus Element In6/1 -> rover_transport/3(udp_write_led)
  Bus Element In2/1 -> rover_bringup/1(foxglove_ws_in)
  Bus Element In5/1 -> rover_bringup/3(diagnostics_agg)
  rover_transport/1(rc_raw_udp) -> Bus Element Out1/1
  rover_transport/3(led_udp) -> Bus Element Out7/1
  rover_bringup/1(foxglove_ws_out) -> Bus Element Out2/1
  rover_bringup/2(teleop_web_cmd_vel_stamped) -> Bus Element Out3/1
  rover_bringup/3(teleop_foxglove_cmd_vel_stamped) -> Bus Element Out4/1
  rover_bringup/4(ui_e_stop_services) -> Bus Element Out5/1

== system RoverPlatformArch/Power ==
  Bus Element In1 : Inport  PortName=battery_udp_data
  rover_battery : Subsystem  mask{design_capacity=40, watchdog_timeout=10}
      settings: PortSchema="{\"entries\":[{\"content\":{\"headerSize\":26,\"margin\":15,\"minimumSpacing\":25,\"sides\":[{\"content\":{\"connectorIds\":[\"In1\"]},\"type\":\"ConnectorPlacement.EquallySpacedRectSide\",\"uuid\":\"6054c9f0-8412-410d-9e26-05323c576afd\"},{\"content\":{\"connectorIds\":[\"Out1\",\"Out2\"],\"side\":\"RIGHT\"},\"type\":\"ConnectorPlacement.EquallySpacedRectSide\",\"uuid\":\"23d80627-c7f5-467f-845e-39a8ba0f8903\"},{\"content\":{\"side\":\"TOP\"},\"type\":\"ConnectorPlacement.EquallySpacedRectSide\",\"uuid\":\"85f79d16-0e4c-46b5-a9e4-5492e918629f\"}]},\"type\":\"ConnectorPlacement.EquallySpacedConnector\",\"uuid\":\"014a8f15-8cf2-4a07-97a2-6bf2fab6c72b\"}],\"packageUris\":[\"http://schema.mathworks.com/mf0/Connector/R2020b\"],\"version\":\"1.0\"}"
  Bus Element Out1 : Outport  PortName=battery_status
  Bus Element Out2 : Outport  Port=2  PortName=diagnostics
  wires:
  rover_battery/1(battery_status) -> Bus Element Out1/1
  Bus Element In1/1 -> rover_battery/1(battery_udp_data)
  rover_battery/2(diagnostics) -> Bus Element Out2/1

== system RoverPlatformArch/RcTransmitter ==
  Bus Element Out1 : Outport  PortName=crsf_udp

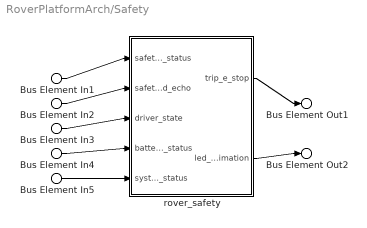
== system RoverPlatformArch/Safety ==
  Bus Element In1 : Inport  PortName=safety_status
  Bus Element In2 : Inport  Port=2  PortName=safety_command_echo
  Bus Element In3 : Inport  Port=3  PortName=driver_state
  Bus Element In4 : Inport  Port=4  PortName=battery_status
  Bus Element In5 : Inport  Port=5  PortName=system_status
  rover_safety : Subsystem  mask{safety_tick_rate=10, battery_temp_critical=50, battery_temp_fatal=60, led_battery_low=0.4, led_battery_critical=0.1}
      settings: PortSchema="{\"entries\":[{\"content\":{\"headerSize\":26,\"margin\":15,\"minimumSpacing\":25,\"sides\":[{\"content\":{\"connectorIds\":[\"In1\",\"In2\",\"In3\",\"In4\",\"In5\"]},\"type\":\"ConnectorPlacement.EquallySpacedRectSide\",\"uuid\":\"6054c9f0-8412-410d-9e26-05323c576afd\"},{\"content\":{\"connectorIds\":[\"Out1\",\"Out2\"],\"side\":\"RIGHT\"},\"type\":\"ConnectorPlacement.EquallySpacedRectSide\",\"uuid\":\"23d80627-c7f5-467f-845e-39a8ba0f8903\"},{\"content\":{\"side\":\"TOP\"},\"type\":\"ConnectorPlacement.EquallySpacedRectSide\",\"uuid\":\"85f79d16-0e4c-46b5-a9e4-5492e918629f\"}]},\"type\":\"ConnectorPlacement.EquallySpacedConnector\",\"uuid\":\"014a8f15-8cf2-4a07-97a2-6bf2fab6c72b\"}],\"packageUris\":[\"http://schema.mathworks.com/mf0/Connector/R2020b\"],\"version\":\"1.0\"}"
  Bus Element Out1 : Outport  PortName=trip_e_stop
  Bus Element Out2 : Outport  Port=2  PortName=led_set_animation
  wires:
  Bus Element In1/1 -> rover_safety/1(safety_status)
  Bus Element In2/1 -> rover_safety/2(safety_command_echo)
  rover_safety/1(trip_e_stop) -> Bus Element Out1/1
  Bus Element In4/1 -> rover_safety/4(battery_status)
  Bus Element In3/1 -> rover_safety/3(driver_state)
  Bus Element In5/1 -> rover_safety/5(system_status)
  rover_safety/2(led_set_animation) -> Bus Element Out2/1

== system RoverPlatformArch/SafetyPlc ==
  Bus Element In1 : Inport  PortName=modbus_coils
  Bus Element Out1 : Outport  PortName=modbus_inputs

== system RoverPlatformArch/SensorPayload ==
  Bus Element Out1 : Outport  PortName=gps_fix

== system RoverPlatformArch/CommandArbitration/rover_crsf_teleop ==
  Bus Element In1 : Inport  PortName=rc_raw_udp
  Bus Element In2 : Inport  Port=2  PortName=safety_status
  Bus Element Out1 : Outport  PortName=teleop_elrs_cmd_vel_stamped
  Bus Element Out2 : Outport  Port=2  PortName=e_stop_services

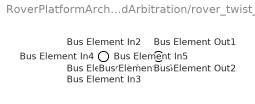
== system RoverPlatformArch/CommandArbitration/rover_twist_mux ==
  Bus Element In1 : Inport  PortName=teleop_elrs_cmd_vel_stamped
  Bus Element In2 : Inport  Port=2  PortName=teleop_driver_interface_cmd_vel_stamped
  Bus Element In3 : Inport  Port=3  PortName=teleop_foxglove_cmd_vel_stamped
  Bus Element In4 : Inport  Port=4  PortName=nav_cmd_vel_stamped
  Bus Element In5 : Inport  Port=5  PortName=safety_status
  Bus Element In6 : Inport  Port=6  PortName=safety_command_echo
  Bus Element Out1 : Outport  PortName=motion_lock
  Bus Element Out2 : Outport  Port=2  PortName=cmd_vel

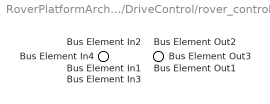
== system RoverPlatformArch/DriveControl/rover_controller ==
  Bus Element In1 : Inport  PortName=cmd_vel
  Bus Element In2 : Inport  Port=2  PortName=wheel_state
  Bus Element In3 : Inport  Port=3  PortName=imu_state
  Bus Element In4 : Inport  Port=4  PortName=robot_description
  Bus Element Out1 : Outport  PortName=wheel_velocity_command
  Bus Element Out2 : Outport  Port=2  PortName=odometry_wheels
  Bus Element Out3 : Outport  Port=3  PortName=imu_data

== system RoverPlatformArch/DriveControl/rover_description ==
  Bus Element Out1 : Outport  PortName=robot_description
  Bus Element Out2 : Outport  Port=2  PortName=tf_static

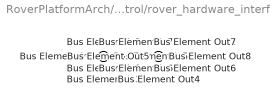
== system RoverPlatformArch/DriveControl/rover_hardware_interface ==
  Bus Element In1 : Inport  PortName=e_stop_services
  Bus Element In2 : Inport  Port=2  PortName=ui_e_stop_services
  Bus Element In3 : Inport  Port=3  PortName=trip_e_stop
  Bus Element In4 : Inport  Port=4  PortName=wheel_velocity_command
  Bus Element In5 : Inport  Port=5  PortName=modbus_inputs
  Bus Element In6 : Inport  Port=6  PortName=encoder_feedback
  Bus Element In7 : Inport  Port=7  PortName=imu_raw
  Bus Element Out1 : Outport  PortName=safety_status
  Bus Element Out2 : Outport  Port=2  PortName=safety_command_echo
  Bus Element Out3 : Outport  Port=3  PortName=driver_state
  Bus Element Out4 : Outport  Port=4  PortName=wheel_state
  Bus Element Out5 : Outport  Port=5  PortName=imu_state
  Bus Element Out6 : Outport  Port=6  PortName=modbus_coils
  Bus Element Out7 : Outport  Port=7  PortName=motor_command
  Bus Element Out8 : Outport  Port=8  PortName=diagnostics

== system RoverPlatformArch/HmiStatus/rover_diag_manager ==
  Bus Element In1 : Inport  PortName=diagnostics
  Bus Element In2 : Inport  Port=2  PortName=diagnostics_from_rover_battery
  Bus Element Out1 : Outport  PortName=system_status
  Bus Element Out2 : Outport  Port=2  PortName=diagnostics_agg

== system RoverPlatformArch/HmiStatus/rover_led ==
  Bus Element In1 : Inport  PortName=led_set_animation
  Bus Element Out1 : Outport  PortName=udp_write_led

== system RoverPlatformArch/Localization/rover_gps_heading ==
  Bus Element In1 : Inport  PortName=gps_fix
  Bus Element In2 : Inport  Port=2  PortName=odom
  Bus Element Out1 : Outport  PortName=gps_heading_imu

== system RoverPlatformArch/Localization/rover_localization ==
  Bus Element In1 : Inport  PortName=tf_static
  Bus Element In2 : Inport  Port=2  PortName=odometry_wheels
  Bus Element In3 : Inport  Port=3  PortName=imu_data
  Bus Element In4 : Inport  Port=4  PortName=gps_fix
  Bus Element In5 : Inport  Port=5  PortName=gps_heading_imu
  Bus Element Out1 : Outport  PortName=odom

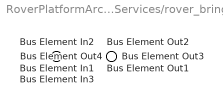
== system RoverPlatformArch/PlatformServices/rover_bringup ==
  Bus Element In1 : Inport  PortName=foxglove_ws_in
  Bus Element In2 : Inport  Port=2  PortName=drive_mode
  Bus Element In3 : Inport  Port=3  PortName=diagnostics_agg
  Bus Element Out1 : Outport  PortName=foxglove_ws_out
  Bus Element Out2 : Outport  Port=2  PortName=teleop_web_cmd_vel_stamped
  Bus Element Out3 : Outport  Port=3  PortName=teleop_foxglove_cmd_vel_stamped
  Bus Element Out4 : Outport  Port=4  PortName=ui_e_stop_services

== system RoverPlatformArch/PlatformServices/rover_msgs ==

== system RoverPlatformArch/PlatformServices/rover_transport ==
  Bus Element In1 : Inport  PortName=crsf_udp
  Bus Element In2 : Inport  Port=2  PortName=bms_udp
  Bus Element In3 : Inport  Port=3  PortName=udp_write_led
  Bus Element Out1 : Outport  PortName=rc_raw_udp
  Bus Element Out2 : Outport  Port=2  PortName=battery_udp_data
  Bus Element Out3 : Outport  Port=3  PortName=led_udp

== system RoverPlatformArch/Power/rover_battery ==
  Bus Element In1 : Inport  PortName=battery_udp_data
  Bus Element Out1 : Outport  PortName=battery_status
  Bus Element Out2 : Outport  Port=2  PortName=diagnostics

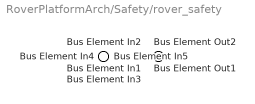
== system RoverPlatformArch/Safety/rover_safety ==
  Bus Element In1 : Inport  PortName=safety_status
  Bus Element In2 : Inport  Port=2  PortName=safety_command_echo
  Bus Element In3 : Inport  Port=3  PortName=driver_state
  Bus Element In4 : Inport  Port=4  PortName=battery_status
  Bus Element In5 : Inport  Port=5  PortName=system_status
  Bus Element Out1 : Outport  PortName=trip_e_stop
  Bus Element Out2 : Outport  Port=2  PortName=led_set_animation
